simulink model "DCDC_Boost_Converter"  (R2024b)
settings: Solver=ode45  StartTime=0.0  StopTime=0.1  RelTol=1e-3
values from neighbouring files (symbols this model uses):
  C_Filter = (I_ripple*Ts)/(8*V_ripple)    (= 1.5625e-05)    [Buck_DCDC_Converter.m]    (also in Buck_DCDC_Converter_Calculation.m = 6.94444444444e-06; DCDC_Boost_Converter_Calculation.m = 2.9296875e-05; DCDC_Buck_Boost_Converter_Calculation.m = 2.9296875e-05)
  D = Vout/Vin    (= 0.4)    [Buck_DCDC_Converter.m]    (also in Buck_DCDC_Converter_Calculation.m = 0.6; DCDC_Boost_Converter_Calculation.m = 0.375; DCDC_Buck_Boost_Converter_Calculation.m = 0.375)
  L_Filter = ((Vin-Vout)*D*Ts)/I_ripple    (= 0.000192)    [Buck_DCDC_Converter.m]    (also in Buck_DCDC_Converter_Calculation.m = 0.000288; DCDC_Boost_Converter_Calculation.m = 0.0012; DCDC_Buck_Boost_Converter_Calculation.m = 0.0012)
  Rload = Vout/Iout    (= 1.6)    [Buck_DCDC_Converter.m]    (also in Buck_DCDC_Converter_Calculation.m = 3.6; DCDC_Boost_Converter_Calculation.m = 25.6; DCDC_Buck_Boost_Converter_Calculation.m = 25.6)
  Ts = 1/Fsw    (= 2e-05)    [Buck_DCDC_Converter.m]    (also in Buck_DCDC_Converter_Calculation.m; DCDC_Boost_Converter_Calculation.m; DCDC_Buck_Boost_Converter_Calculation.m)
  Vin = 100    [Buck_DCDC_Converter.m]    (also in Buck_DCDC_Converter_Calculation.m; DCDC_Boost_Converter_Calculation.m; DCDC_Buck_Boost_Converter_Calculation.m)
  Vout = 40    [Buck_DCDC_Converter.m]    (also in Buck_DCDC_Converter_Calculation.m = 60; DCDC_Boost_Converter_Calculation.m = 160; DCDC_Buck_Boost_Converter_Calculation.m = 160)
libraries: spsCurrentMeasurementLib x3, spsSeriesRLCBranchLib x3, spsVoltageMeasurementLib x3, spsDCVoltageSourceLib x1, spsDiodeLib x1, spsMosfetLib x1, slpidlib x1, spsPWMGeneratorDCDCLib x1, sps_lib x1
settings Model: Creator=SUDHAK1  LastModifiedBy=SUDHAK1

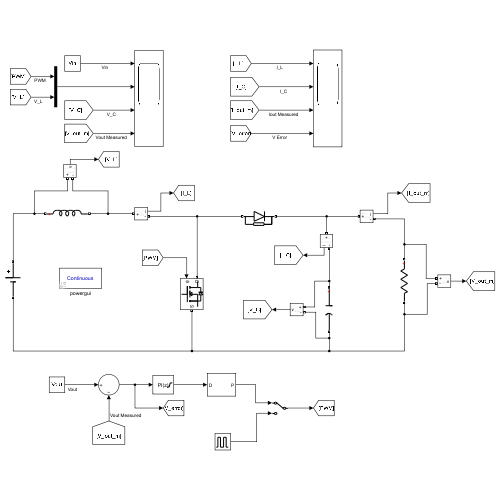
[thumbnail: Simulink's stored preview of the top-level diagram]
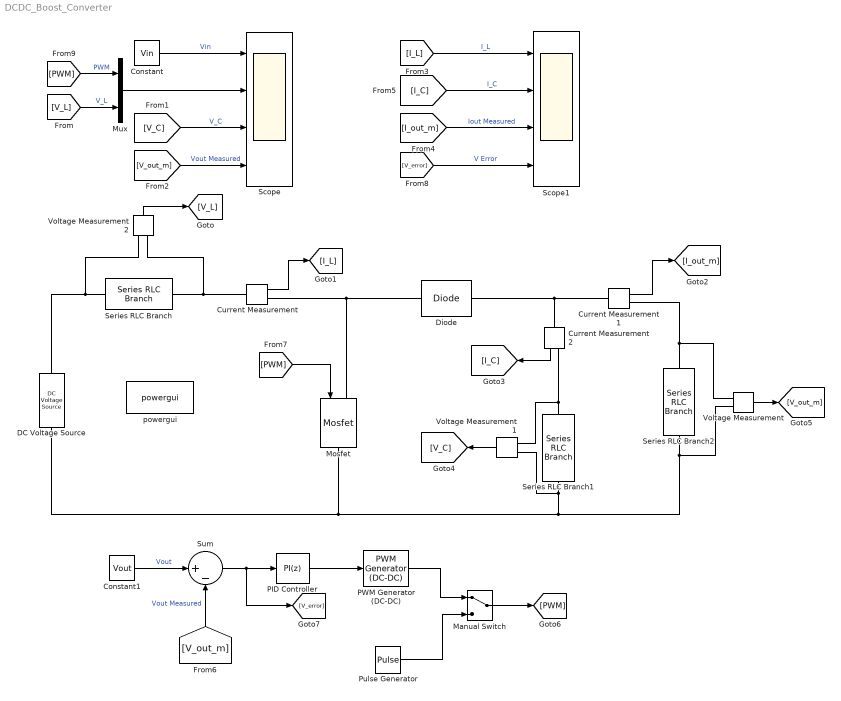
== system DCDC_Boost_Converter ==
  Constant : Constant  Value=Vin
  Constant1 : Constant  Value=Vout
  Current Measurement : spsCurrentMeasurementLib/Current Measurement  PhasorSimulation=off  OutputType=Complex  PSBequivalent=0
  Current Measurement1 : spsCurrentMeasurementLib/Current Measurement  PhasorSimulation=off  OutputType=Complex  PSBequivalent=0
  Current Measurement2 : spsCurrentMeasurementLib/Current Measurement  PhasorSimulation=off  OutputType=Complex  PSBequivalent=0
  DC Voltage Source : spsDCVoltageSourceLib/DC Voltage Source  Amplitude=Vin  Measurements=None
  Diode : spsDiodeLib/Diode  Ron=0.0001  Lon=0  Vf=0.8  IC=0  UseSnubber=0  Rs=500  Cs=250e-9  Measurements=off
  Manual Switch : ManualSwitch
  Mosfet : spsMosfetLib/Mosfet  Ron=0.0001  Lon=0  Rd=0.0001  Vfd=0  IC=0  Rs=1e5  Cs=inf  Measurements=off
  Mux : Mux  Inputs=2
  PID Controller : slpidlib/PID Controller  Controller=PI  Form=Parallel  TimeDomain=Discrete-time  UseExternalTs=off  SampleTime=-1  IntegratorMethod=Forward Euler  FilterMethod=Forward Euler  ControllerParametersSource=internal  P=1  I=1  UseKiTs=off  D=0  UseExternalDerivativeSource=off  N=100  UseFilter=on  TunerSelectOption=Transfer Function Based (PID Tuner App)  InitialConditionSource=internal  InitialConditionForIntegrator=0  InitialConditionForFilter=0  DifferentiatorICPrevScaledInput=0  ExternalReset=none  TrackingMode=off  Kt=1  LimitOutput=on  SatLimitsSource=internal  UpperSaturationLimit=100  LowerSaturationLimit=0  LinearizeAsGain=off  AntiWindupMode=none  Kb=1  LimitIntegrator=off  UpperIntegratorSaturationLimit=inf  LowerIntegratorSaturationLimit=-inf  POutMin=[]  POutMax=[]  IOutMin=[]  IOutMax=[]  DOutMin=[]  DOutMax=[]  NOutMin=[]  NOutMax=[]  SumOutMin=[]  SumOutMax=[]  SaturationOutMin=[]  SaturationOutMax=[]  PParamMin=[]  PParamMax=[]  IParamMin=[]  IParamMax=[]  DParamMin=[]  DParamMax=[]  NParamMin=[]  NParamMax=[]  KbParamMin=[]  KbParamMax=[]  KtParamMin=[]  KtParamMax=[]  KbOutMin=[]  KbOutMax=[]  KtOutMin=[]  KtOutMax=[]  IntegratorOutMin=[]  IntegratorOutMax=[]  FilterOutMin=[]  FilterOutMax=[]  SumI1OutMin=[]  SumI1OutMax=[]  SumI2OutMin=[]  SumI2OutMax=[]  SumI3OutMin=[]  SumI3OutMax=[]  SumI4OutMin=[]  SumI4OutMax=[]  SumDOutMin=[]  SumDOutMax=[]  DifferentiatorOutMin=[]  DifferentiatorOutMax=[]  FilterDiffOutCoefMin=[]  FilterDiffOutCoefMax=[]  ReciprocalOutMin=[]  ReciprocalOutMax=[]  SumDenOutMin=[]  SumDenOutMax=[]  SumNumOutMin=[]  SumNumOutMax=[]  DivideOutMin=[]  DivideOutMax=[]  UdiffTsProdOutMin=[]  UdiffTsProdOutMax=[]  NTsProdOutMin=[]  NTsProdOutMax=[]  UintegralTsProdOutMin=[]  UintegralTsProdOutMax=[]  UngainTsProdOutMin=[]  UngainTsProdOutMax=[]  ClampingZeroOutDataTypeStr=Inherit: Inherit via back propagation  ClampingZeroOutMin=[]  ClampingZeroOutMax=[]  FilterDenConstantOutDataTypeStr=Inherit: Inherit via back propagation  FilterDenConstantOutMin=[]  FilterDenConstantOutMax=[]  PCopyOutDataTypeStr=Inherit: Inherit via back propagation  PCopyOutMin=[]  PCopyOutMax=[]  NCopyOutDataTypeStr=Inherit: Inherit via back propagation  NCopyOutMin=[]  NCopyOutMax=[]  IntegratorContinuousStateAttributes=''  IntegratorStateMustResolveToSignalObject=off  IntegratorRTWStateStorageClass=Auto  FilterContinuousStateAttributes=''  FilterStateMustResolveToSignalObject=off  FilterRTWStateStorageClass=Auto  ParallelPVariant=InternalParameters  IdealPVariant=Disabled  IVariant=InternalParameters  DVariant=Disabled  IntegratorVariant=Discrete  SatVariant=Enabled  AWVariant=Passthrough  PCopyVariant=Disabled  TRVariant=Disabled  FdbkBlocksVariant=Forward  IdealPFdbkVariant=Disabled  SatFdbkVariant=Disabled  DerivativeFilterVariant=Disabled  NVariant=Disabled  NCopyVariant=Disabled_SignalSpec  FilterICVariant=Disabled  IntegratorICVariant=InternalICs  ExternalResetVariant=Disabled  TRSumVariant=Passthrough  SumFdbkVariant=Disabled  SumVariant=Sum_PI  TsampFilterVariant=InternalTs  TsampNgainVariant=Passthrough  TsampIntegralVariant=Disabled_SignalSpec  ExternalSaturationOutDataTypeStr=Inherit: Same as second input  DerivativeSourceVariant=Disabled  PreIntVariant=InternalPreInt
  PWM Generator (DC-DC) : spsPWMGeneratorDCDCLib/PWM Generator (DC-DC)  Fsw=Fsw  Ts=0
  Pulse Generator : DiscretePulseGenerator  PulseType=Time based  Period=Ts  PulseWidth=D*100
  Scope : Scope  NumInputPorts=4
  Scope1 : Scope  NumInputPorts=4
  Series RLC Branch : spsSeriesRLCBranchLib/Series RLC Branch  LConnTagsString=__new0  RConnTagsString=__new0  BranchType=L  Resistance=1  Inductance=L_Filter  SetiL0=off  InitialCurrent=0  Capacitance=1e-6  Setx0=off  InitialVoltage=0  Measurements=None
  Series RLC Branch1 : spsSeriesRLCBranchLib/Series RLC Branch  LConnTagsString=__new0  RConnTagsString=__new0  BranchType=C  Resistance=1  Inductance=1e-3  SetiL0=off  InitialCurrent=0  Capacitance=C_Filter  Setx0=off  InitialVoltage=0  Measurements=None
  Series RLC Branch2 : spsSeriesRLCBranchLib/Series RLC Branch  LConnTagsString=__new0  RConnTagsString=__new0  BranchType=R  Resistance=Rload  Inductance=1e-3  SetiL0=off  InitialCurrent=0  Capacitance=1e-6  Setx0=off  InitialVoltage=0  Measurements=None
  Sum : Sum  Inputs=|+-
  Voltage Measurement : spsVoltageMeasurementLib/Voltage Measurement  PhasorSimulation=off  OutputType=Complex  PSBequivalent=0
  Voltage Measurement1 : spsVoltageMeasurementLib/Voltage Measurement  PhasorSimulation=off  OutputType=Complex  PSBequivalent=0
  Voltage Measurement2 : spsVoltageMeasurementLib/Voltage Measurement  PhasorSimulation=off  OutputType=Complex  PSBequivalent=0
  powergui : sps_lib/powergui  Priority=1  SimulationMode=Continuous  SampleTime=50e-6  frequency=60  Iterations=50  frequencyindice=0  Pbase=100e6  ErrMax=1e-4  UnitsV=kV  UnitsW=MW  buscounter=0  FunctionMessages=off  echomessages=off  EnableUseOfTLC=off  CurrentSourceSwitches=off  DisableSnubberDevices=off  DisableRonSwitches=off  DisableVfSwitches=off  DisplayEquations=off  AutomaticDiscreteSolvers=off  SolverType=Tustin/Backward Euler (TBE)  Interpol=off  ExternalGateDelay=off  methode=off  Ts=100  x0status=blocks  SPID=on  SwTol=0  HookPort=off  NonlinearTolerance=1e-4  nMaxIteration=100  ContinueOnMaxIteration=off  RestoreLinks=warning  ResistiveCurrentMeasurement=off  Frange=[0:2:500]  Ylog=off  Xlog=on  ShowGrid=off  save=off  variable=ZData  structure=0  ZoomFFT=off  StartTime=0.0  cycles=1  DisplayStyle=1  fundamental=60  FreqAxis=off  MaxFrequency=1000  frequencyindicesteady=1  RmsSteady=1  display=off
  wires:
  [PWM] -> Mosfet/1
  Constant1/1 -> Sum/1  "Vout"
  [V_error] -> Scope1/4  "V Error"
  [I_C] -> Scope1/2  "I_C"
  Mux/1 -> Scope/2
  [V_out_m] -> Scope/4  "Vout Measured"
  [V_out_m] -> Sum/2  "Vout Measured"
  PID Controller/1 -> PWM Generator (DC-DC)/1
  Constant/1 -> Scope/1  "Vin"
  Voltage Measurement/1 -> [V_out_m]
  Current Measurement1/1 -> [I_out_m]
  [I_out_m] -> Scope1/3  "Iout Measured"
  [I_L] -> Scope1/1  "I_L"
  Voltage Measurement1/1 -> [V_C]
  Voltage Measurement2/1 -> [V_L]
  [V_C] -> Scope/3  "V_C"
  Current Measurement2/1 -> [I_C]
  Sum/1 -> [V_error], PID Controller/1
  Current Measurement/1 -> [I_L]
  Pulse Generator/1 -> Manual Switch/2
  PWM Generator (DC-DC)/1 -> Manual Switch/1
  Manual Switch/1 -> [PWM]
  [PWM] -> Mux/1  "PWM"
  [V_L] -> Mux/2  "V_L"
  connections:
  Series RLC Branch2/RConn1 -- Mosfet/RConn1 -- DC Voltage Source/LConn1 -- Voltage Measurement1/LConn2 -- Series RLC Branch1/RConn1 -- Voltage Measurement/LConn2
  Voltage Measurement2/LConn2 -- Series RLC Branch/RConn1 -- Current Measurement/LConn1
  Series RLC Branch2/LConn1 -- Current Measurement1/RConn1 -- Voltage Measurement/LConn1
  Series RLC Branch/LConn1 -- Voltage Measurement2/LConn1 -- DC Voltage Source/RConn1
  Series RLC Branch1/LConn1 -- Current Measurement2/RConn1 -- Voltage Measurement1/LConn1
  Diode/LConn1 -- Mosfet/LConn1 -- Current Measurement/RConn1
  Diode/RConn1 -- Current Measurement1/LConn1 -- Current Measurement2/LConn1
